simulink model "boost_cascade_pi_mrac_mf_sps"  (R2025a)
settings: Solver=ode23tb  StartTime=0.0  StopTime=0.5  MaxStep=5e-06  RelTol=1e-05
PreLoadFcn:
  | if ~exist('BM', 'var'), boost_mrac_params; end
InitFcn:
  | if ~exist('BM', 'var'), boost_mrac_params; end
undefined symbols (not defined in the file): BM, DiscIntNeverNeededParam
libraries: spsSeriesRLCBranchLib x5, spsIdealSwitchLib x2, spsDiodeLib x1, spsMosfetLib x1, spsControlledVoltageSourceLib x1, spsCurrentMeasurementLib x1, spsVoltageMeasurementLib x1, simulink x1, sps_lib x1
Description:
  | DC-DC boost converter, cascade PI-based MRAC, outer loop tracks the reference-model output (model-following variant), circuit model (Specialized Power Systems). Recreation of Yanarates & Zhou, IEEE Access 10 (2022) 44909. Parameters: struct BM from boost_mrac_params.m.
settings Model: Creator=runner  LastModifiedBy=runner
settings DataIOCC: SaveOutput=off  SignalLogging=off  SaveTime=off
settings DebuggingCC: AlgebraicLoopMsg=error

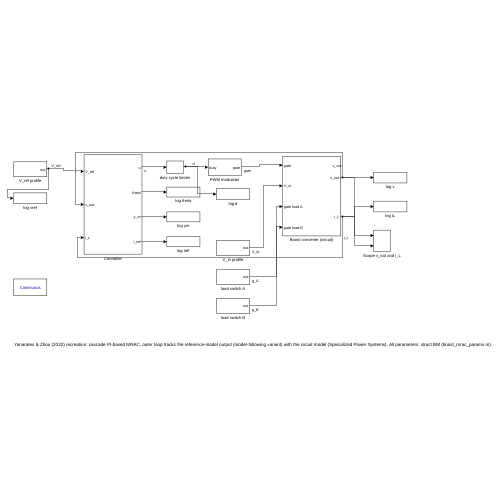
[thumbnail: Simulink's stored preview of the top-level diagram]
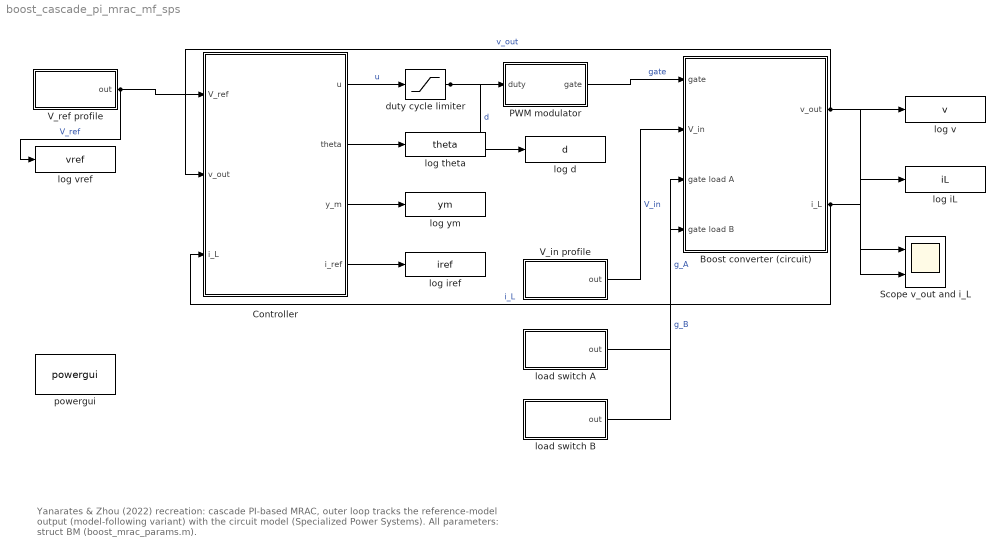
== system boost_cascade_pi_mrac_mf_sps ==
  note: Yanarates & Zhou (2022) recreation: cascade PI-based MRAC, outer loop tracks the reference-model output (model-following variant) with the circuit model (Specialized Power Systems). All parameters: struct BM (boost_mrac_params.m).
  Boost converter (circuit) : Subsystem
  Controller : Subsystem
  PWM modulator : Subsystem
  Scope v_out and i_L : Scope  NumInputPorts=2
  V_in profile : Subsystem
  V_ref profile : Subsystem
  duty cycle limiter : Saturate  UpperLimit=BM.dmax  LowerLimit=BM.dmin
  load switch A : Subsystem
  load switch B : Subsystem
  log d : ToWorkspace  VariableName=d  SaveFormat=Timeseries  SampleTime=BM.Ts
  log iL : ToWorkspace  VariableName=iL  SaveFormat=Timeseries  SampleTime=BM.Ts
  log iref : ToWorkspace  VariableName=iref  SaveFormat=Timeseries  SampleTime=BM.Ts
  log theta : ToWorkspace  VariableName=theta  SaveFormat=Timeseries  SampleTime=BM.Ts
  log v : ToWorkspace  VariableName=v  SaveFormat=Timeseries  SampleTime=BM.Ts
  log vref : ToWorkspace  VariableName=vref  SaveFormat=Timeseries  SampleTime=BM.Ts
  log ym : ToWorkspace  VariableName=ym  SaveFormat=Timeseries  SampleTime=BM.Ts
  powergui : sps_lib/powergui  Priority=1  SimulationMode=Continuous  SampleTime=50e-6  frequency=60  Iterations=50  frequencyindice=0  Pbase=100e6  ErrMax=1e-4  UnitsV=kV  UnitsW=MW  buscounter=0  FunctionMessages=off  echomessages=off  EnableUseOfTLC=off  CurrentSourceSwitches=off  DisableSnubberDevices=off  DisableRonSwitches=off  DisableVfSwitches=off  DisplayEquations=off  AutomaticDiscreteSolvers=off  SolverType=Tustin/Backward Euler (TBE)  Interpol=off  ExternalGateDelay=off  methode=off  Ts=100  x0status=blocks  SPID=on  SwTol=0  HookPort=off  NonlinearTolerance=1e-4  nMaxIteration=100  ContinueOnMaxIteration=off  RestoreLinks=warning  ResistiveCurrentMeasurement=off  Frange=[0:2:500]  Ylog=off  Xlog=on  ShowGrid=off  save=off  variable=ZData  structure=0  ZoomFFT=off  StartTime=0.0  cycles=1  DisplayStyle=1  fundamental=60  FreqAxis=off  MaxFrequency=1000  frequencyindicesteady=1  RmsSteady=1  display=off
  wires:
  V_ref profile/1(out) -> Controller/1(V_ref), log vref/1  "V_ref"
  Controller/1(u) -> duty cycle limiter/1  "u"
  duty cycle limiter/1 -> PWM modulator/1(duty), log d/1  "d"
  PWM modulator/1(gate) -> Boost converter (circuit)/1(gate)  "gate"
  V_in profile/1(out) -> Boost converter (circuit)/2(V_in)  "V_in"
  load switch A/1(out) -> Boost converter (circuit)/3(gate load A)  "g_A"
  load switch B/1(out) -> Boost converter (circuit)/4(gate load B)  "g_B"
  Boost converter (circuit)/1(v_out) -> Controller/2(v_out), log v/1, Scope v_out and i_L/1  "v_out"
  Boost converter (circuit)/2(i_L) -> Controller/3(i_L), log iL/1, Scope v_out and i_L/2  "i_L"
  Controller/2(theta) -> log theta/1
  Controller/3(y_m) -> log ym/1
  Controller/4(i_ref) -> log iref/1

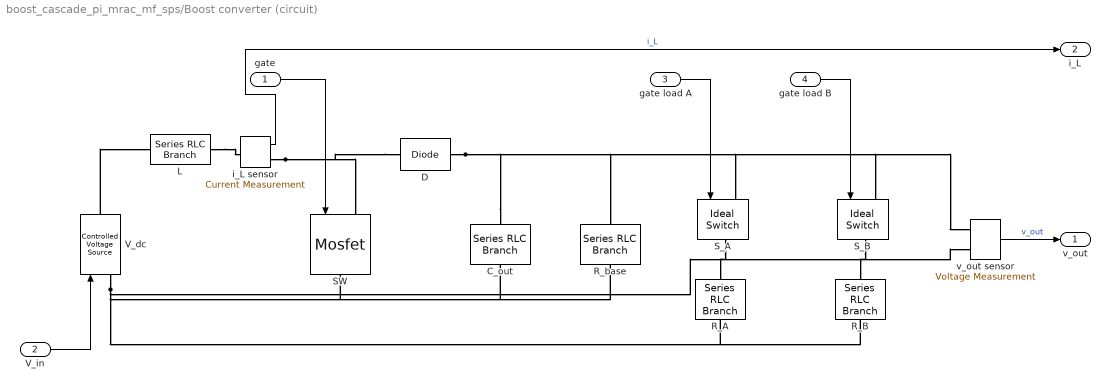
== system boost_cascade_pi_mrac_mf_sps/Boost converter (circuit) ==
  gate : Inport
  V_in : Inport  Port=2
  gate load A : Inport  Port=3
  gate load B : Inport  Port=4
  C_out : spsSeriesRLCBranchLib/Series RLC Branch  LConnTagsString=__new0  RConnTagsString=__new0  BranchType=C  Resistance=1  Inductance=1e-3  SetiL0=off  InitialCurrent=0  Capacitance=BM.C  Setx0=on  InitialVoltage=BM.v0  Measurements=None
  D : spsDiodeLib/Diode  Ron=BM.Ron_d  Lon=0  Vf=BM.Vf_d  IC=0  UseSnubber=0  Rs=inf  Cs=0  Measurements=off
  L : spsSeriesRLCBranchLib/Series RLC Branch  LConnTagsString=__new0  RConnTagsString=__new0  BranchType=L  Resistance=1  Inductance=BM.L  SetiL0=on  InitialCurrent=BM.iL0  Capacitance=1e-6  Setx0=off  InitialVoltage=0  Measurements=None
  R_A : spsSeriesRLCBranchLib/Series RLC Branch  LConnTagsString=__new0  RConnTagsString=__new0  BranchType=R  Resistance=BM.R_a  Inductance=1e-3  SetiL0=off  InitialCurrent=0  Capacitance=1e-6  Setx0=off  InitialVoltage=0  Measurements=None
  R_B : spsSeriesRLCBranchLib/Series RLC Branch  LConnTagsString=__new0  RConnTagsString=__new0  BranchType=R  Resistance=BM.R_b  Inductance=1e-3  SetiL0=off  InitialCurrent=0  Capacitance=1e-6  Setx0=off  InitialVoltage=0  Measurements=None
  R_base : spsSeriesRLCBranchLib/Series RLC Branch  LConnTagsString=__new0  RConnTagsString=__new0  BranchType=R  Resistance=BM.R_base  Inductance=1e-3  SetiL0=off  InitialCurrent=0  Capacitance=1e-6  Setx0=off  InitialVoltage=0  Measurements=None
  SW : spsMosfetLib/Mosfet  Ron=BM.Ron_sw  Lon=0  Rd=0.01  Vfd=0  IC=0  Rs=1e5  Cs=inf  Measurements=off
  S_A : spsIdealSwitchLib/Ideal Switch  Ron=1e-3  Lon=0  IC=0  Rs=1e5  Cs=inf  Measurements=off
  S_B : spsIdealSwitchLib/Ideal Switch  Ron=1e-3  Lon=0  IC=0  Rs=1e5  Cs=inf  Measurements=off
  V_dc : spsControlledVoltageSourceLib/Controlled Voltage Source  Initialize=on  Source_Type=DC  Amplitude=BM.vin(1)  Phase=0  Frequency=0  Measurements=None
  i_L sensor : spsCurrentMeasurementLib/Current Measurement  PhasorSimulation=off  OutputType=Complex  PSBequivalent=0
  v_out sensor : spsVoltageMeasurementLib/Voltage Measurement  PhasorSimulation=off  OutputType=Complex  PSBequivalent=0
  v_out : Outport
  i_L : Outport  Port=2
  wires:
  V_in/1 -> V_dc/1
  gate/1 -> SW/1
  gate load A/1 -> S_A/1
  gate load B/1 -> S_B/1
  i_L sensor/1 -> i_L/1  "i_L"
  v_out sensor/1 -> v_out/1  "v_out"
  connections:
  V_dc/RConn1 -- L/LConn1
  L/RConn1 -- i_L sensor/LConn1
  D/LConn1 -- i_L sensor/RConn1 -- SW/LConn1
  C_out/LConn1 -- D/RConn1 -- R_base/LConn1 -- S_A/LConn1 -- S_B/LConn1 -- v_out sensor/LConn1
  S_A/RConn1 -- R_A/LConn1
  S_B/RConn1 -- R_B/LConn1
  SW/RConn1 -- V_dc/LConn1 -- C_out/RConn1 -- R_base/RConn1 -- R_A/RConn1 -- R_B/RConn1 -- v_out sensor/LConn2

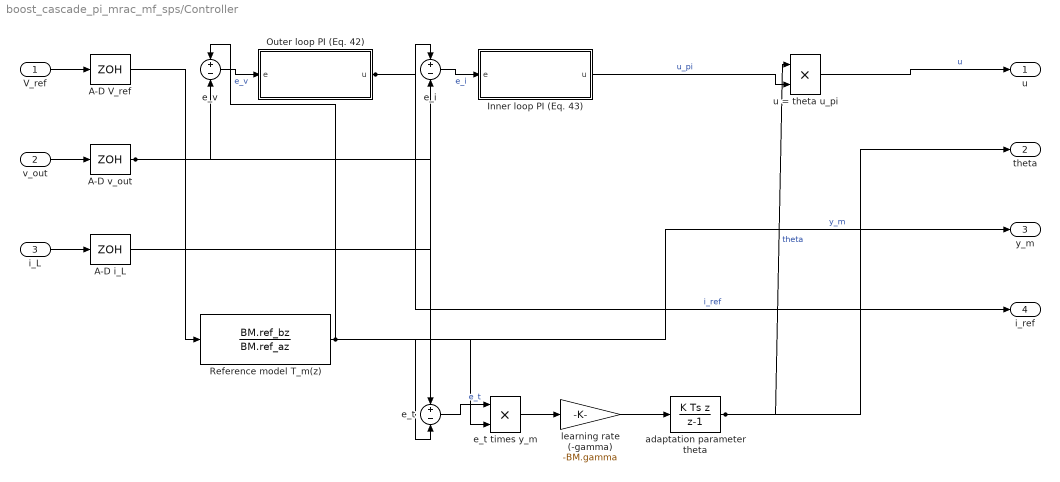
== system boost_cascade_pi_mrac_mf_sps/Controller ==
  V_ref : Inport
  v_out : Inport  Port=2
  i_L : Inport  Port=3
  A-D V_ref : ZeroOrderHold  SampleTime=BM.Ts
  A-D i_L : ZeroOrderHold  SampleTime=BM.Ts
  A-D v_out : ZeroOrderHold  SampleTime=BM.Ts
  Inner loop PI (Eq. 43) : Subsystem
  Outer loop PI (Eq. 42) : Subsystem
  Reference model T_m(z) : DiscreteTransferFcn  Numerator=BM.ref_bz  Denominator=BM.ref_az  SampleTime=BM.Ts
  adaptation parameter theta : DiscreteIntegrator  IntegratorMethod=Integration: Backward Euler  gainval=1  InitialCondition=BM.theta0  SampleTime=BM.Ts  ICPrevOutput=DiscIntNeverNeededParam  ICPrevScaledInput=DiscIntNeverNeededParam
  e_i : Sum  Inputs=+-
  e_t : Sum  Inputs=+-
  e_t times y_m : Product  Inputs=**
  e_v : Sum  Inputs=+-
  learning rate (-gamma) : Gain  Gain=-BM.gamma
  u = theta u_pi : Product  Inputs=**
  u : Outport
  theta : Outport  Port=2
  y_m : Outport  Port=3
  i_ref : Outport  Port=4
  wires:
  V_ref/1 -> A-D V_ref/1
  v_out/1 -> A-D v_out/1
  i_L/1 -> A-D i_L/1
  A-D v_out/1 -> e_v/2, e_t/1
  e_v/1 -> Outer loop PI (Eq. 42)/1(e)  "e_v"
  Outer loop PI (Eq. 42)/1(u) -> e_i/1, i_ref/1  "i_ref"
  A-D i_L/1 -> e_i/2
  e_i/1 -> Inner loop PI (Eq. 43)/1(e)  "e_i"
  A-D V_ref/1 -> Reference model T_m(z)/1
  Reference model T_m(z)/1 -> e_v/1, e_t/2, e_t times y_m/2, y_m/1  "y_m"
  e_t/1 -> e_t times y_m/1  "e_t"
  e_t times y_m/1 -> learning rate (-gamma)/1
  learning rate (-gamma)/1 -> adaptation parameter theta/1
  adaptation parameter theta/1 -> u = theta u_pi/1, theta/1  "theta"
  Inner loop PI (Eq. 43)/1(u) -> u = theta u_pi/2  "u_pi"
  u = theta u_pi/1 -> u/1  "u"

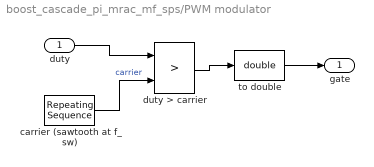
== system boost_cascade_pi_mrac_mf_sps/PWM modulator ==
  duty : Inport
  carrier (sawtooth at f_sw) : simulink/Sources/Repeating Sequence  rep_seq_t=[0 BM.Tsw]  rep_seq_y=[0 1]
  duty > carrier : RelationalOperator  Operator=>  OutDataTypeStr=boolean  RndMeth=Simplest  InputSameDT=off
  to double : DataTypeConversion  OutDataTypeStr=double  SaturateOnIntegerOverflow=off  RndMeth=Floor
  gate : Outport
  wires:
  duty/1 -> duty > carrier/1
  carrier (sawtooth at f_sw)/1 -> duty > carrier/2  "carrier"
  duty > carrier/1 -> to double/1
  to double/1 -> gate/1

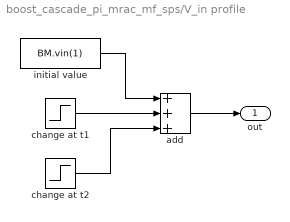
== system boost_cascade_pi_mrac_mf_sps/V_in profile ==
  add : Sum  Inputs=+++
  change at t1 : Step  Time=BM.t_vin(1)  After=BM.vin(2)-BM.vin(1)  SampleTime=0
  change at t2 : Step  Time=BM.t_vin(2)  After=BM.vin(3)-BM.vin(2)  SampleTime=0
  initial value : Constant  Value=BM.vin(1)
  out : Outport
  wires:
  initial value/1 -> add/1
  change at t1/1 -> add/2
  change at t2/1 -> add/3
  add/1 -> out/1

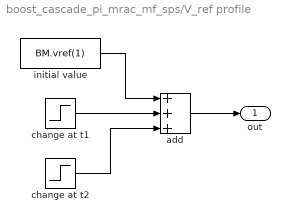
== system boost_cascade_pi_mrac_mf_sps/V_ref profile ==
  add : Sum  Inputs=+++
  change at t1 : Step  Time=BM.t_vref(1)  After=BM.vref(2)-BM.vref(1)  SampleTime=0
  change at t2 : Step  Time=BM.t_vref(2)  After=BM.vref(3)-BM.vref(2)  SampleTime=0
  initial value : Constant  Value=BM.vref(1)
  out : Outport
  wires:
  initial value/1 -> add/1
  change at t1/1 -> add/2
  change at t2/1 -> add/3
  add/1 -> out/1

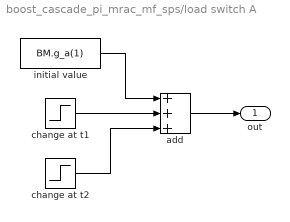
== system boost_cascade_pi_mrac_mf_sps/load switch A ==
  add : Sum  Inputs=+++
  change at t1 : Step  Time=BM.t_rload(1)  After=BM.g_a(2)-BM.g_a(1)  SampleTime=0
  change at t2 : Step  Time=BM.t_rload(2)  After=BM.g_a(3)-BM.g_a(2)  SampleTime=0
  initial value : Constant  Value=BM.g_a(1)
  out : Outport
  wires:
  initial value/1 -> add/1
  change at t1/1 -> add/2
  change at t2/1 -> add/3
  add/1 -> out/1

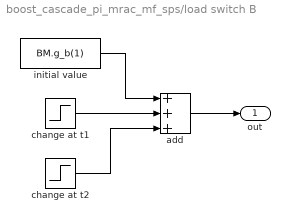
== system boost_cascade_pi_mrac_mf_sps/load switch B ==
  add : Sum  Inputs=+++
  change at t1 : Step  Time=BM.t_rload(1)  After=BM.g_b(2)-BM.g_b(1)  SampleTime=0
  change at t2 : Step  Time=BM.t_rload(2)  After=BM.g_b(3)-BM.g_b(2)  SampleTime=0
  initial value : Constant  Value=BM.g_b(1)
  out : Outport
  wires:
  initial value/1 -> add/1
  change at t1/1 -> add/2
  change at t2/1 -> add/3
  add/1 -> out/1

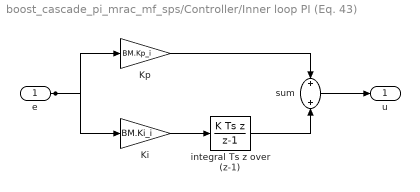
== system boost_cascade_pi_mrac_mf_sps/Controller/Inner loop PI (Eq. 43) ==
  e : Inport
  Ki : Gain  Gain=BM.Ki_i
  Kp : Gain  Gain=BM.Kp_i
  integral Ts z over (z-1) : DiscreteIntegrator  IntegratorMethod=Integration: Backward Euler  gainval=1  SampleTime=BM.Ts  ICPrevOutput=DiscIntNeverNeededParam  ICPrevScaledInput=DiscIntNeverNeededParam
  sum : Sum
  u : Outport
  wires:
  e/1 -> Kp/1, Ki/1
  Ki/1 -> integral Ts z over (z-1)/1
  Kp/1 -> sum/1
  integral Ts z over (z-1)/1 -> sum/2
  sum/1 -> u/1

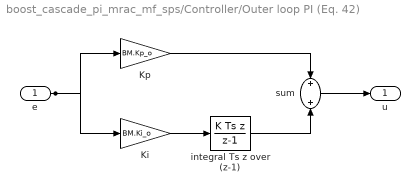
== system boost_cascade_pi_mrac_mf_sps/Controller/Outer loop PI (Eq. 42) ==
  e : Inport
  Ki : Gain  Gain=BM.Ki_o
  Kp : Gain  Gain=BM.Kp_o
  integral Ts z over (z-1) : DiscreteIntegrator  IntegratorMethod=Integration: Backward Euler  gainval=1  SampleTime=BM.Ts  ICPrevOutput=DiscIntNeverNeededParam  ICPrevScaledInput=DiscIntNeverNeededParam
  sum : Sum
  u : Outport
  wires:
  e/1 -> Kp/1, Ki/1
  Ki/1 -> integral Ts z over (z-1)/1
  Kp/1 -> sum/1
  integral Ts z over (z-1)/1 -> sum/2
  sum/1 -> u/1
